simulink model "Inverter_pq_comp_sat_sim"  (R2023b)
settings: Solver=FixedStepDiscrete  StartTime=0.0  StopTime=2  RelTol=1e-3  EnableMultiTasking=on
InitFcn:
  | %% Definition of the parameters
  | 
  | Parameter_Definition
  | 
  | %% Damping
  | 
  | Rd = 3.9;
  | 
  | %% PRes Gains Calculation
  | 
  | % Definicao das grandezas
  | w_cl = 1j*2*pi*1200;  % Phase Crossing Frequency
  | no   = 1;           % Integral Resonant Constant
  | A    = 1;             % Carrier Amplitude
  | 
  | % Kp calculation
  | a0 = 1;
  | a1 = Rd*Cf;
  | b0 = 0;
  | b1 = Lf+Lg;
  | b2 = Rd*Lf*Cf+Rd*Lg*Cf;
  | b3 = Lf*Lg*Cf;
  | 
  | G_lcl = (a1*w_cl+a0)/(b3*w_cl^3+b2*w_cl^2+b1*w_cl+b0);
  | % G_lcl = 1/((Lf+Lg)*w_cl+Rf);
  | 
  | G_PWM = (1/A)*(1-w_cl*Ts/4)/(1+w_cl*Ts/4);
  | 
  | G_wc  = (Vdc/2)*(1/I_base)*G_lcl*G_PWM;
  | 
  | G_wc_abs = abs(G_wc);
  | 
  | Kp = 1/G_wc_abs;
  | 
  | % Discretized Controller Gains
  | ressonance_list = [1,5,7,11,13];
  | 
  | n_res = length(ressonance_list);
  | a = zeros(2,n_res);
  | b = zeros(2,n_res);
  | Ki_res = zeros(1,n_res);
  | 
  | % for i = 1:n_res
  | %   k = ressonance_list(i);
  | %   Ki_res(i) = (2.2*Kp)/(no*T_gr);
  | %   a(i) = (2*Ki_res(i)*Ts)/(4+((k*w_gr)^2)*Ts^2);
  | %   b(i) = (-8+2*((k*w_gr)^2)*Ts^2)/(4+((k*w_gr)^2)*Ts^2);
  | % end
  | 
  | % wc is the cutoff frequency/damping factor in rad/s
  | wc = 2;
  | 
  | for i = 1:n_res
  |   k = ressonance_list(i);
  |   wk = k * w_gr; % Resonant frequency for this harmonic
  | 
  |   Ki_res(i) = (2.2*Kp)/(0.8*no*T_gr);
  | 
  |   % 1. Calculate the common denominator
  |   den = 4 + 4*wc*Ts + (wk^2)*(Ts^2);
  | ... (+14 lines)
values from neighbouring files (symbols this model uses):
  a1_sogi = single(2*(w0_sogi^2-c_sogi^2)/den0_sogi)    [Parameter_Definition.m]
  a2_sogi = single((c_sogi^2                 - k_sogi*w0_sogi*c_sogi                 + w0_sogi^2)/den0_sogi)    [Parameter_Definition.m]
  bD_sogi = single(k_sogi*w0_sogi*c_sogi/den0_sogi)    [Parameter_Definition.m]
  bQ_sogi = single(k_sogi*w0_sogi^2/den0_sogi)    [Parameter_Definition.m]
  Cdc = 1.5e-3    (= 0.0015)    [Parameter_Definition.m]
  Cf = 5e-6    (= 5e-06)    [Parameter_Definition.m]
  f_gr = 60    [Parameter_Definition.m]
  I_base = S_base/(sqrt(3)*V_gr)    [Parameter_Definition.m]
  Lf = 1e-3    (= 0.001)    [Parameter_Definition.m]
  Lg = 0.5e-3    (= 0.0005)    [Parameter_Definition.m]
  Rdc = 0.1/(2*pi*60*Cdc)    (= 0.176838825658)    [Parameter_Definition.m]
  Rf = 0.1*Xf    (= 0.0376991118431)    [Parameter_Definition.m]
  Rg = 0.1*Xg    (= 0.0188495559215)    [Parameter_Definition.m]
  S_base = S_rated    (= 1000)    [Parameter_Definition.m]
  Ts = 2*(4167)/100e6    (= 8.334e-05)    [Parameter_Definition.m]
  Tstep = Ts/1000    (= 8.334e-08)    [Parameter_Definition.m]
  V_base = sqrt(3)*V_gr    [Parameter_Definition.m]
  V_gr = 127    [Parameter_Definition.m]
  Vdc = 800    [Parameter_Definition.m]
  Vdc_base = Vdc    (= 800)    [Parameter_Definition.m]
  w_gr = 2*pi*f_gr    (= 376.991118431)    [Parameter_Definition.m]
undefined symbols (not defined in the file or in its folder): gH_LUT, gQ_LUT, gV_LUT, lH_vetor, lQ_vetor, lV_vetor
libraries: spsSeriesRLCBranchLib x22, spsIGBTDiodeLib x12, spsCurrentMeasurementLib x9, spsVoltageMeasurementLib x5, c2837xDlib x4, spsACVoltageSourceLib x3, spsGroundLib x3, spsDCVoltageSourceLib x2, spsTriangleGeneratorLib x1, simulink x1, eeRmsMeasurement x1, spsTHDLib x1
(part 3 of 3)

== matlab function Inverter_pq_comp_sat_sim/RMS_fcn1 ==
  data: RMSin input; yout output
function yout = fcn(RMSin)

win = 200;

persistent sampleRMS
    if isempty(sampleRMS)
        sampleRMS = single(0.0);
    end
    if sampleRMS>=win
        sampleRMS = single(0.0);
    end

persistent RMSout
if isempty(RMSout)
    RMSout = single(0.0);
end    
persistent sumRMS
if isempty(sumRMS)
    sumRMS = single(0.0);
end
persistent RMSinArray
     if isempty(RMSinArray)
         RMSinArray = zeros(1,win);
     end

sampleRMS = sampleRMS + 1;      

%RMS of Input Signal
sumRMS = sumRMS + RMSin*RMSin - RMSinArray(1,sampleRMS);
RMSinArray(1,sampleRMS) = RMSin*RMSin;
if sumRMS>=0.0
    RMSout = sqrt(sumRMS/win);
end

%RMSout = RMSout_temp;

yout = RMSout;

== matlab function Inverter_pq_comp_sat_sim/RMS_fcn2 ==
  data: RMSin input; yout output
function yout = fcn(RMSin)

win = 200;

persistent sampleRMS
    if isempty(sampleRMS)
        sampleRMS = single(0.0);
    end
    if sampleRMS>=win
        sampleRMS = single(0.0);
    end

persistent RMSout
if isempty(RMSout)
    RMSout = single(0.0);
end    
persistent sumRMS
if isempty(sumRMS)
    sumRMS = single(0.0);
end
persistent RMSinArray
     if isempty(RMSinArray)
         RMSinArray = zeros(1,win);
     end

sampleRMS = sampleRMS + 1;      

%RMS of Input Signal
sumRMS = sumRMS + RMSin*RMSin - RMSinArray(1,sampleRMS);
RMSinArray(1,sampleRMS) = RMSin*RMSin;
if sumRMS>=0.0
    RMSout = sqrt(sumRMS/win);
end

%RMSout = RMSout_temp;

yout = RMSout;

== matlab function Inverter_pq_comp_sat_sim/RMS_fcn3 ==
  data: RMSin input; yout output
function yout = fcn(RMSin)

win = 200;

persistent sampleRMS
    if isempty(sampleRMS)
        sampleRMS = single(0.0);
    end
    if sampleRMS>=win
        sampleRMS = single(0.0);
    end

persistent RMSout
if isempty(RMSout)
    RMSout = single(0.0);
end    
persistent sumRMS
if isempty(sumRMS)
    sumRMS = single(0.0);
end
persistent RMSinArray
     if isempty(RMSinArray)
         RMSinArray = zeros(1,win);
     end

sampleRMS = sampleRMS + 1;      

%RMS of Input Signal
sumRMS = sumRMS + RMSin*RMSin - RMSinArray(1,sampleRMS);
RMSinArray(1,sampleRMS) = RMSin*RMSin;
if sumRMS>=0.0
    RMSout = sqrt(sumRMS/win);
end

%RMSout = RMSout_temp;

yout = RMSout;
